simulink model "sschdlexViennaRectifierModel"  (R2026a)
settings: Solver=FixedStepDiscrete  StopTime=0.8  MaxStep=1e-4
PreLoadFcn:
  | % Copyright 2017-2023 The MathWorks, Inc.
  | 
  | %% System Parameters
  | Vs    = 120*sqrt(3); % AC source line-to-line (V, rms)
  | Vpeak = Vs/sqrt(3)*sqrt(2); % AC source line-to-ground (V, peak)
  | R = 0.1;  % Resistance (Ohm)
  | L = 2e-3; % Inductance (H)
  | Vdcnom = 400;  % Nominal output dc voltage (V)
  | Pnom   = 10e3; % Nominal power (W)
  | Imax   = Pnom/(1.5*Vpeak); % Maximum ac current        (A)
  | Inom   = Pnom/Vdcnom;      % Nominal output dc current (A)
  | Iload  = 0.2*Inom;         % Initial load current      (A)
  | 
  | %% Control Parameters
  | fsw = 5e3;        % Switching frequency (Hz)
  | Ts  = 1/(50*fsw); % Fundamental sample time (s)
  | Tsc = 1/(10*fsw); % Control sample time (s)
  | 
  | Kp_vdc = 0.7386; % Proportional gain dc-link voltage controller
  | Ki_vdc = 135.6;  % Integral gain dc-link voltage controller
  | Kp_id  = 8.407;  % Proportional gain d-axis current controller
  | Ki_id  = 1127;   % Integral gain d-axis current controller
  | Kp_iq  = 11.91;  % Proportional gain q-axis current controller
  | Ki_iq  = 3706;   % Integral gain q-axis current controller
  | Kp_vn  = 0.4912; % Proportional gain neutral voltage controller
libraries: ee_lib x27, nesl_utility x13, fl_lib x10, eeTransforms x4, slpidlib x4, eeGeneralControl x4, eePwmGeneratorViennaRectifier x1, eeSinusoidalMeasurement x1, eePowerMeasurement x1
(part 1 of 2)
CloseFcn:
  | try,close(h1_ee_vienna_rectifier),end
  | clear h1_ee_vienna_rectifier
  | 
  | clear simlog_ee_vienna_rectifier
  | clear logsout_ee_vienna_rectifier
  | 
  | clear Vs Vpeak R L Vdcnom Pnom Imax Inom Iload
  | clear fsw Ts Tsc Kp_vdc Ki_vdc Kp_id Ki_id Kp_iq Ki_iq Kp_vn
Description:
  | Vienna Rectifier Control
settings Model: DataTypeOverride=Off  Creator=The MathWorks, Inc.  LastModifiedBy=The MathWorks, Inc.
settings DataIOCC: SignalLoggingName=logsout_ee_vienna_rectifier
settings OptimizationCC: ConditionallyExecuteInputs=off
settings DebuggingCC: AlgebraicLoopMsg=error  UnderspecifiedInitializationDetection=Classic  SingleTaskRateTransMsg=error  PregeneratedLibrarySubsystemCodeDiagnostic=none
settings HardwareCC: ProdHWDeviceType=ASIC/FPGA->ASIC/FPGA  TargetBitPerLong=64.0  TargetBitPerPointer=64.0  TargetBitPerSizeT=64.0  TargetBitPerPtrDiffT=64.0  TargetLongLongMode=on  TargetIntDivRoundTo=Zero  TargetEndianess=LittleEndian  TargetWordSize=64.0  TargetHWDeviceType=Custom Processor->MATLAB Host Computer  ProdEqTarget=off
settings SimscapeCC: SimscapeNormalizeSystem=off  SimscapeNominalValues="[{\"value\":\"1\",\"unit\":\"A\"},{\"value\":\"1\",\"unit\":\"bar\"},{\"value\":\"1\",\"unit\":\"cm^2\"},{\"value\":\"1\",\"unit\":\"cm^3/s\"},{\"value\":\"1\",\"unit\":\"kJ/kg\"},{\"value\":\"1\",\"unit\":\"kW\"},{\"value\":\"1\",\"unit\":\"l\"},{\"value\":\"1\",\"unit\":\"N\"},{\"value\":\"1\",\"unit\":\"N*m\"},{\"value\":\"1\",\"unit\":\"V\"}]"  SimscapeLogName=simlog_ee_vienna_rectifier  SimscapeLogDataHistory=200000.0

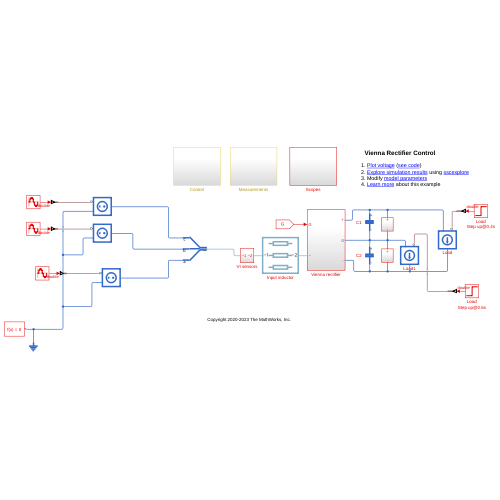
[thumbnail: Simulink's stored preview of the top-level diagram]
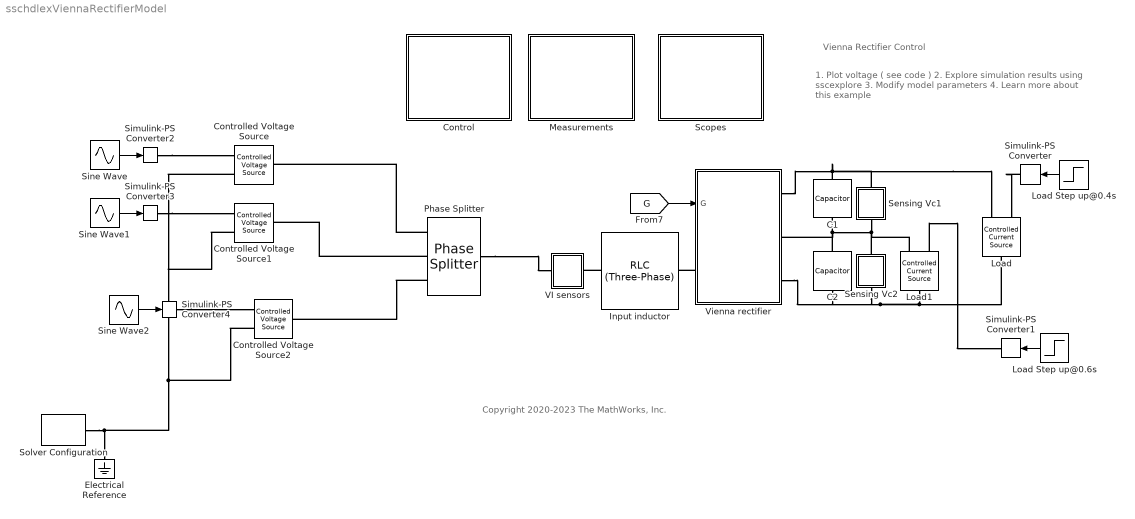
== system sschdlexViennaRectifierModel ==
  note: Copyright 2020-2023 The MathWorks, Inc.
  note: Vienna Rectifier Control
  note: 1. Plot voltage ( see code )
      | 2. Explore simulation results using sscexplore
      | 3. Modify model parameters
      | 4. Learn more about this example
  C1 : fl_lib/Electrical/Electrical Elements/Capacitor  c=2000e-6 F  r=1e-5 Ohm  g=0 1/Ohm  i_specify=off  i_priority=None  i=0 A  i_nominal_specify=off  i_nominal_value=1  i_nominal_unit=A  v_specify=off  v_priority=None  v=0 V  v_nominal_specify=off  v_nominal_value=1  v_nominal_unit=V  vc_specify=off  vc_priority=High  vc=0 V  vc_nominal_specify=off  vc_nominal_value=1  vc_nominal_unit=V
  C2 : fl_lib/Electrical/Electrical Elements/Capacitor  c=2000e-6 F  r=1e-5 Ohm  g=0 1/Ohm  i_specify=off  i_priority=None  i=0 A  i_nominal_specify=off  i_nominal_value=1  i_nominal_unit=A  v_specify=off  v_priority=None  v=0 V  v_nominal_specify=off  v_nominal_value=1  v_nominal_unit=V  vc_specify=off  vc_priority=High  vc=0 V  vc_nominal_specify=off  vc_nominal_value=1  vc_nominal_unit=V
  Control : Subsystem
  Controlled Voltage Source : fl_lib/Electrical/Electrical Sources/Controlled Voltage Source
  Controlled Voltage Source1 : fl_lib/Electrical/Electrical Sources/Controlled Voltage Source
  Controlled Voltage Source2 : fl_lib/Electrical/Electrical Sources/Controlled Voltage Source
  Electrical Reference : fl_lib/Electrical/Electrical Elements/Electrical Reference
  Input inductor : ee_lib/Passive/RLC Assemblies/RLC (Three-Phase)  port_option=ee.enum.threePhasePort.composite  component_structure=4  R=R Ohm  L=L H  C=1e-6 F  R_parasitic=1e-6 Ohm  G_parasitic=1e-6 1/Ohm  IL_specify=off  IL_priority=High  IL=[ 0 0 0 ] A  IL_nominal_specify=off  IL_nominal_value=1  IL_nominal_unit=A  VC_specify=off  VC_priority=High  VC=[ 0 0 0 ] V  VC_nominal_specify=off  VC_nominal_value=1  VC_nominal_unit=V
  Load : fl_lib/Electrical/Electrical Sources/Controlled Current Source
  Load Step up@0.4s : Step  Time=0.4  InitialValue=Iload  FinalValue=Inom  SampleTime=Ts
  Load Step up@0.6s : Step  Time=0.6  FinalValue=2  SampleTime=Ts
  Load1 : fl_lib/Electrical/Electrical Sources/Controlled Current Source
  Measurements : Subsystem
  Phase Splitter : ee_lib/Connectors & References/Phase Splitter
  Scopes : Subsystem
  Sensing Vc1 : Subsystem
  Sensing Vc2 : Subsystem
  Simulink-PS Converter{,1..4} (5 alike) : nesl_utility/Simulink-PS Converter  PhysicalDomain=network_engine_domain  SubClassName=ps_input  LeftPortType=input  RightPortType=output  PseudoPeriodic=off  Frequencies=[]  NoiseDistribution=none  NoiseParameters=[]  Unit=1  AffineConversion=off  FilteringAndDerivatives=provide  SimscapeFilterOrder=1  InputFilterTimeConstant=0.001  UdotUserProvided=0
  Sine Wave : Sin  Amplitude=Vs/sqrt(2)  Frequency=2*pi*60  Phase=2*pi/3  SampleTime=Ts
  Sine Wave1 : Sin  Amplitude=Vs/sqrt(2)  Frequency=2*pi*60  Phase=4*pi/3  SampleTime=Ts
  Sine Wave2 : Sin  Amplitude=Vs/sqrt(2)  Frequency=2*pi*60  SampleTime=Ts
  Solver Configuration : nesl_utility/Solver Configuration  PhysicalDomain=network_engine_domain  SubClassName=solver  LeftPortType=input  RightPortType=generic  Tones=[]  Harmonics=[]  SimulateNoise=off  Profile=off  UseLocalSampling=off  EnableSwitchedLinearOptims=on  FrequencyDomain=off  UseCCode=off  RelTol=0.001  AbsTol=1e-06  MinStep=1e-09  ToWorkspace=off  RevertToSquareIcSolve=off  NumHomotopyIterations=100  PhasorMode=off  PhasorModeNumHarmonics=1  ConsistencySolver=NEWTON_FTOL  CanonicalOrdering=UNORDERED  OptimizeIntermediates=UNOPTIMIZED  IndexReductionMethod=DerivativeReplacement  DoDC=off  ResidualTolerance=1e-09  ConsistencyTolSource=GLOBAL  ConsistencyAbsTol=0.001  ConsistencyRelTol=0.001  ConsistencyTolFactor=0.001  UseLocalSolver=on  LocalSolverChoice=NE_BACKWARD_EULER_ADVANCER  ResolveIndetEquations=on  FunctionEvalNumThread=1  LocalSolverSampleTime=Ts  DoFixedCost=off  MaxNonlinIter=4  MaxModeIter=2  ComputeImpulses=off  ImpulseIterations=2  LinearAlgebra=auto  LinearAlgebraNumThread=0  EquationFormulation=NE_TIME_EF  DelaysMemoryBudget=1024  AutomaticFiltering=on  FilteringTimeConstant=0.001  PartitionStorageMethod=AS_NEEDED  PartitionMemoryBudget=1024  PartitionMethod=FAST  MultibodyUseLocalSolver=off  MultibodyLocalSolverChoice=ODE1  MultibodyLocalSolverSampleTime=0.001
  VI sensors : Subsystem
  Vienna rectifier : Subsystem
  wires:
  Load Step up@0.4s/1 -> Simulink-PS Converter/1
  [G] -> Vienna rectifier/1(G)
  Load Step up@0.6s/1 -> Simulink-PS Converter1/1
  Sine Wave/1 -> Simulink-PS Converter2/1
  Sine Wave1/1 -> Simulink-PS Converter3/1
  Sine Wave2/1 -> Simulink-PS Converter4/1
  connections:
  C1/RConn1 -- C2/LConn1 -- Vienna rectifier/RConn2 -- Load1/RConn2 -- Sensing Vc2/LConn1 -- Sensing Vc1/RConn1
  Vienna rectifier/RConn1 -- C1/LConn1 -- Sensing Vc1/LConn1 -- Load/RConn2
  Solver Configuration/RConn1 -- Controlled Voltage Source2/RConn2 -- Controlled Voltage Source1/RConn2 -- Controlled Voltage Source/RConn2 -- Electrical Reference/LConn1
  Sensing Vc2/RConn1 -- C2/RConn1 -- Vienna rectifier/RConn3 -- Load1/LConn1 -- Load/LConn1
  Phase Splitter/LConn1 -- VI sensors/LConn1
  Simulink-PS Converter/RConn1 -- Load/RConn1
  Input inductor/LConn1 -- VI sensors/RConn1
  Vienna rectifier/LConn1 -- Input inductor/RConn1
  Load1/RConn1 -- Simulink-PS Converter1/RConn1
  Simulink-PS Converter2/RConn1 -- Controlled Voltage Source/RConn1
  Simulink-PS Converter3/RConn1 -- Controlled Voltage Source1/RConn1
  Simulink-PS Converter4/RConn1 -- Controlled Voltage Source2/RConn1
  Phase Splitter/RConn3 -- Controlled Voltage Source/LConn1
  Phase Splitter/RConn2 -- Controlled Voltage Source1/LConn1
  Phase Splitter/RConn1 -- Controlled Voltage Source2/LConn1

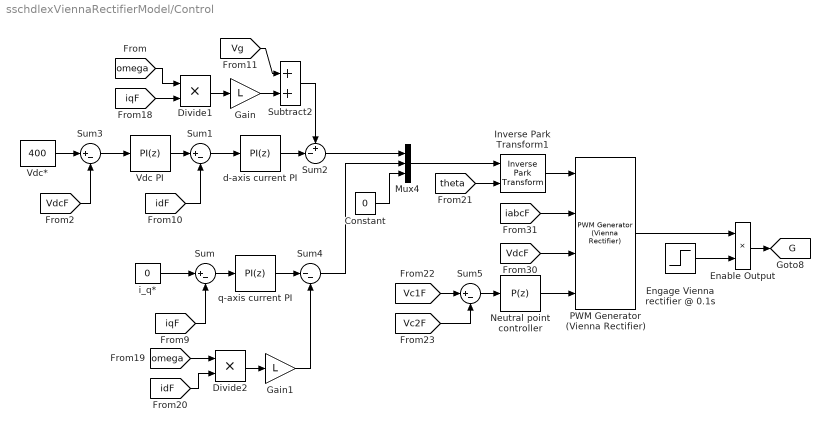
== system sschdlexViennaRectifierModel/Control ==
  Constant : Constant  Value=0  SampleTime=Tsc
  Divide1 : Product  Inputs=**
  Divide2 : Product  Inputs=**
  Enable Output : Product
  Engage Vienna rectifier @ 0.1s : Step  Time=0.1  SampleTime=Ts
  Gain : Gain  Gain=L
  Gain1 : Gain  Gain=L
  Inverse Park Transform1 : eeTransforms/Inverse Park Transform  AxisAlignment=Q-axis  PowerInvariant=off
  Mux4 : Mux  Inputs=3
  Neutral point controller : slpidlib/PID Controller  Controller=P  Form=Parallel  TimeDomain=Discrete-time  UseExternalTs=off  SampleTime=-1  IntegratorMethod=Forward Euler  FilterMethod=Forward Euler  ControllerParametersSource=internal  P=Kp_vn  I=80/2  UseKiTs=off  D=0  UseExternalDerivativeSource=off  N=100  UseFilter=on  TunerSelectOption=Transfer Function Based (PID Tuner App)  InitialConditionSource=internal  InitialConditionForIntegrator=0  InitialConditionForFilter=0  DifferentiatorICPrevScaledInput=0  ExternalReset=none  TrackingMode=off  Kt=1  LimitOutput=on  SatLimitsSource=internal  UpperSaturationLimit=1  LowerSaturationLimit=-1  LinearizeAsGain=on  AntiWindupMode=back-calculation  Kb=1000  LimitIntegrator=off  UpperIntegratorSaturationLimit=inf  LowerIntegratorSaturationLimit=-inf  POutMin=[]  POutMax=[]  IOutMin=[]  IOutMax=[]  DOutMin=[]  DOutMax=[]  NOutMin=[]  NOutMax=[]  SumOutMin=[]  SumOutMax=[]  SaturationOutMin=[]  SaturationOutMax=[]  PParamMin=[]  PParamMax=[]  IParamMin=[]  IParamMax=[]  DParamMin=[]  DParamMax=[]  NParamMin=[]  NParamMax=[]  KbParamMin=[]  KbParamMax=[]  KtParamMin=[]  KtParamMax=[]  KbOutMin=[]  KbOutMax=[]  KtOutMin=[]  KtOutMax=[]  IntegratorOutMin=[]  IntegratorOutMax=[]  FilterOutMin=[]  FilterOutMax=[]  SumI1OutMin=[]  SumI1OutMax=[]  SumI2OutMin=[]  SumI2OutMax=[]  SumI3OutMin=[]  SumI3OutMax=[]  SumI4OutMin=[]  SumI4OutMax=[]  SumDOutMin=[]  SumDOutMax=[]  DifferentiatorOutMin=[]  DifferentiatorOutMax=[]  FilterDiffOutCoefMin=[]  FilterDiffOutCoefMax=[]  ReciprocalOutMin=[]  ReciprocalOutMax=[]  SumDenOutMin=[]  SumDenOutMax=[]  SumNumOutMin=[]  SumNumOutMax=[]  DivideOutMin=[]  DivideOutMax=[]  UdiffTsProdOutMin=[]  UdiffTsProdOutMax=[]  NTsProdOutMin=[]  NTsProdOutMax=[]  UintegralTsProdOutMin=[]  UintegralTsProdOutMax=[]  UngainTsProdOutMin=[]  UngainTsProdOutMax=[]  ClampingZeroOutDataTypeStr=Inherit: Inherit via back propagation  ClampingZeroOutMin=[]  ClampingZeroOutMax=[]  FilterDenConstantOutDataTypeStr=Inherit: Inherit via back propagation  FilterDenConstantOutMin=[]  FilterDenConstantOutMax=[]  PCopyOutDataTypeStr=Inherit: Inherit via back propagation  PCopyOutMin=[]  PCopyOutMax=[]  NCopyOutDataTypeStr=Inherit: Inherit via back propagation  NCopyOutMin=[]  NCopyOutMax=[]  IntegratorContinuousStateAttributes=''  IntegratorStateMustResolveToSignalObject=off  IntegratorRTWStateStorageClass=Auto  FilterContinuousStateAttributes=''  FilterStateMustResolveToSignalObject=off  FilterRTWStateStorageClass=Auto  ParallelPVariant=InternalParameters  IdealPVariant=Disabled  IVariant=Disabled  DVariant=Disabled  IntegratorVariant=Disabled  SatVariant=Enabled  AWVariant=Disabled  PCopyVariant=Disabled  TRVariant=Disabled  FdbkBlocksVariant=Forward  IdealPFdbkVariant=Disabled  SatFdbkVariant=Disabled  DerivativeFilterVariant=Disabled  NVariant=Disabled  NCopyVariant=Disabled_SignalSpec  FilterICVariant=Disabled  IntegratorICVariant=Disabled  ExternalResetVariant=Disabled  TRSumVariant=Passthrough  SumFdbkVariant=Disabled  SumVariant=Passthrough_P  TsampFilterVariant=InternalTs  TsampNgainVariant=Passthrough  TsampIntegralVariant=Disabled_SignalSpec  ExternalSaturationOutDataTypeStr=Inherit: Same as second input  DerivativeSourceVariant=Disabled  PreIntVariant=InternalPreInt
  PWM Generator (Vienna Rectifier) : eePwmGeneratorViennaRectifier/PWM Generator (Vienna Rectifier)  fsw=fsw  Ts=Ts
      settings: SamplingMode=Asymmetric
  Subtract2 : Sum
  Sum{,1,3,5} (4 alike) : Sum  Inputs=|+-
  Sum2 : Sum  Inputs=+-|
  Sum4 : Sum  Inputs=|--
  Vdc PI : slpidlib/PID Controller  Controller=PI  Form=Parallel  TimeDomain=Discrete-time  UseExternalTs=off  SampleTime=Tsc  IntegratorMethod=Forward Euler  FilterMethod=Forward Euler  ControllerParametersSource=internal  P=Kp_vdc  I=Ki_vdc  UseKiTs=off  D=0  UseExternalDerivativeSource=off  N=100  UseFilter=on  TunerSelectOption=Transfer Function Based (PID Tuner App)  InitialConditionSource=internal  InitialConditionForIntegrator=0  InitialConditionForFilter=0  DifferentiatorICPrevScaledInput=0  ExternalReset=none  TrackingMode=off  Kt=1  LimitOutput=on  SatLimitsSource=internal  UpperSaturationLimit=1.5*Imax  LowerSaturationLimit=-1.5*Imax  LinearizeAsGain=on  AntiWindupMode=back-calculation  Kb=1000  LimitIntegrator=off  UpperIntegratorSaturationLimit=inf  LowerIntegratorSaturationLimit=-inf  POutMin=[]  POutMax=[]  IOutMin=[]  IOutMax=[]  DOutMin=[]  DOutMax=[]  NOutMin=[]  NOutMax=[]  SumOutMin=[]  SumOutMax=[]  SaturationOutMin=[]  SaturationOutMax=[]  PParamMin=[]  PParamMax=[]  IParamMin=[]  IParamMax=[]  DParamMin=[]  DParamMax=[]  NParamMin=[]  NParamMax=[]  KbParamMin=[]  KbParamMax=[]  KtParamMin=[]  KtParamMax=[]  KbOutMin=[]  KbOutMax=[]  KtOutMin=[]  KtOutMax=[]  IntegratorOutMin=[]  IntegratorOutMax=[]  FilterOutMin=[]  FilterOutMax=[]  SumI1OutMin=[]  SumI1OutMax=[]  SumI2OutMin=[]  SumI2OutMax=[]  SumI3OutMin=[]  SumI3OutMax=[]  SumI4OutMin=[]  SumI4OutMax=[]  SumDOutMin=[]  SumDOutMax=[]  DifferentiatorOutMin=[]  DifferentiatorOutMax=[]  FilterDiffOutCoefMin=[]  FilterDiffOutCoefMax=[]  ReciprocalOutMin=[]  ReciprocalOutMax=[]  SumDenOutMin=[]  SumDenOutMax=[]  SumNumOutMin=[]  SumNumOutMax=[]  DivideOutMin=[]  DivideOutMax=[]  UdiffTsProdOutMin=[]  UdiffTsProdOutMax=[]  NTsProdOutMin=[]  NTsProdOutMax=[]  UintegralTsProdOutMin=[]  UintegralTsProdOutMax=[]  UngainTsProdOutMin=[]  UngainTsProdOutMax=[]  ClampingZeroOutDataTypeStr=Inherit: Inherit via back propagation  ClampingZeroOutMin=[]  ClampingZeroOutMax=[]  FilterDenConstantOutDataTypeStr=Inherit: Inherit via back propagation  FilterDenConstantOutMin=[]  FilterDenConstantOutMax=[]  PCopyOutDataTypeStr=Inherit: Inherit via back propagation  PCopyOutMin=[]  PCopyOutMax=[]  NCopyOutDataTypeStr=Inherit: Inherit via back propagation  NCopyOutMin=[]  NCopyOutMax=[]  IntegratorContinuousStateAttributes=''  IntegratorStateMustResolveToSignalObject=off  IntegratorRTWStateStorageClass=Auto  FilterContinuousStateAttributes=''  FilterStateMustResolveToSignalObject=off  FilterRTWStateStorageClass=Auto  ParallelPVariant=InternalParameters  IdealPVariant=Disabled  IVariant=InternalParameters  DVariant=Disabled  IntegratorVariant=Discrete  SatVariant=Enabled  AWVariant=BackCalculation  PCopyVariant=Disabled  TRVariant=Disabled  FdbkBlocksVariant=Forward  IdealPFdbkVariant=Disabled  SatFdbkVariant=Disabled  DerivativeFilterVariant=Disabled  NVariant=Disabled  NCopyVariant=Disabled_SignalSpec  FilterICVariant=Disabled  IntegratorICVariant=InternalICs  ExternalResetVariant=Disabled  TRSumVariant=Passthrough  SumFdbkVariant=Disabled  SumVariant=Sum_PI  TsampFilterVariant=InternalTs  TsampNgainVariant=Passthrough  TsampIntegralVariant=Disabled_SignalSpec  ExternalSaturationOutDataTypeStr=Inherit: Same as second input  DerivativeSourceVariant=Disabled  PreIntVariant=InternalPreInt
  Vdc* : Constant  Value=400  SampleTime=Tsc
  d-axis current PI : slpidlib/PID Controller  Controller=PI  Form=Parallel  TimeDomain=Discrete-time  UseExternalTs=off  SampleTime=Tsc  IntegratorMethod=Forward Euler  FilterMethod=Forward Euler  ControllerParametersSource=internal  P=Kp_id  I=Ki_id  UseKiTs=off  D=0  UseExternalDerivativeSource=off  N=100  UseFilter=on  TunerSelectOption=Transfer Function Based (PID Tuner App)  InitialConditionSource=internal  InitialConditionForIntegrator=0  InitialConditionForFilter=0  DifferentiatorICPrevScaledInput=0  ExternalReset=none  TrackingMode=off  Kt=1  LimitOutput=on  SatLimitsSource=internal  UpperSaturationLimit=R*Imax*2  LowerSaturationLimit=-R*Imax*2  LinearizeAsGain=on  AntiWindupMode=back-calculation  Kb=1000  LimitIntegrator=off  UpperIntegratorSaturationLimit=inf  LowerIntegratorSaturationLimit=-inf  POutMin=[]  POutMax=[]  IOutMin=[]  IOutMax=[]  DOutMin=[]  DOutMax=[]  NOutMin=[]  NOutMax=[]  SumOutMin=[]  SumOutMax=[]  SaturationOutMin=[]  SaturationOutMax=[]  PParamMin=[]  PParamMax=[]  IParamMin=[]  IParamMax=[]  DParamMin=[]  DParamMax=[]  NParamMin=[]  NParamMax=[]  KbParamMin=[]  KbParamMax=[]  KtParamMin=[]  KtParamMax=[]  KbOutMin=[]  KbOutMax=[]  KtOutMin=[]  KtOutMax=[]  IntegratorOutMin=[]  IntegratorOutMax=[]  FilterOutMin=[]  FilterOutMax=[]  SumI1OutMin=[]  SumI1OutMax=[]  SumI2OutMin=[]  SumI2OutMax=[]  SumI3OutMin=[]  SumI3OutMax=[]  SumI4OutMin=[]  SumI4OutMax=[]  SumDOutMin=[]  SumDOutMax=[]  DifferentiatorOutMin=[]  DifferentiatorOutMax=[]  FilterDiffOutCoefMin=[]  FilterDiffOutCoefMax=[]  ReciprocalOutMin=[]  ReciprocalOutMax=[]  SumDenOutMin=[]  SumDenOutMax=[]  SumNumOutMin=[]  SumNumOutMax=[]  DivideOutMin=[]  DivideOutMax=[]  UdiffTsProdOutMin=[]  UdiffTsProdOutMax=[]  NTsProdOutMin=[]  NTsProdOutMax=[]  UintegralTsProdOutMin=[]  UintegralTsProdOutMax=[]  UngainTsProdOutMin=[]  UngainTsProdOutMax=[]  ClampingZeroOutDataTypeStr=Inherit: Inherit via back propagation  ClampingZeroOutMin=[]  ClampingZeroOutMax=[]  FilterDenConstantOutDataTypeStr=Inherit: Inherit via back propagation  FilterDenConstantOutMin=[]  FilterDenConstantOutMax=[]  PCopyOutDataTypeStr=Inherit: Inherit via back propagation  PCopyOutMin=[]  PCopyOutMax=[]  NCopyOutDataTypeStr=Inherit: Inherit via back propagation  NCopyOutMin=[]  NCopyOutMax=[]  IntegratorContinuousStateAttributes=''  IntegratorStateMustResolveToSignalObject=off  IntegratorRTWStateStorageClass=Auto  FilterContinuousStateAttributes=''  FilterStateMustResolveToSignalObject=off  FilterRTWStateStorageClass=Auto  ParallelPVariant=InternalParameters  IdealPVariant=Disabled  IVariant=InternalParameters  DVariant=Disabled  IntegratorVariant=Discrete  SatVariant=Enabled  AWVariant=BackCalculation  PCopyVariant=Disabled  TRVariant=Disabled  FdbkBlocksVariant=Forward  IdealPFdbkVariant=Disabled  SatFdbkVariant=Disabled  DerivativeFilterVariant=Disabled  NVariant=Disabled  NCopyVariant=Disabled_SignalSpec  FilterICVariant=Disabled  IntegratorICVariant=InternalICs  ExternalResetVariant=Disabled  TRSumVariant=Passthrough  SumFdbkVariant=Disabled  SumVariant=Sum_PI  TsampFilterVariant=InternalTs  TsampNgainVariant=Passthrough  TsampIntegralVariant=Disabled_SignalSpec  ExternalSaturationOutDataTypeStr=Inherit: Same as second input  DerivativeSourceVariant=Disabled  PreIntVariant=InternalPreInt
  i_q* : Constant  Value=0  SampleTime=Tsc
  q-axis current PI : slpidlib/PID Controller  Controller=PI  Form=Parallel  TimeDomain=Discrete-time  UseExternalTs=off  SampleTime=Tsc  IntegratorMethod=Forward Euler  FilterMethod=Forward Euler  ControllerParametersSource=internal  P=Kp_iq  I=Ki_iq  UseKiTs=off  D=0  UseExternalDerivativeSource=off  N=100  UseFilter=on  TunerSelectOption=Transfer Function Based (PID Tuner App)  InitialConditionSource=internal  InitialConditionForIntegrator=0  InitialConditionForFilter=0  DifferentiatorICPrevScaledInput=0  ExternalReset=none  TrackingMode=off  Kt=1  LimitOutput=on  SatLimitsSource=internal  UpperSaturationLimit=R*Imax*2  LowerSaturationLimit=-R*Imax*2  LinearizeAsGain=on  AntiWindupMode=back-calculation  Kb=1000  LimitIntegrator=off  UpperIntegratorSaturationLimit=inf  LowerIntegratorSaturationLimit=-inf  POutMin=[]  POutMax=[]  IOutMin=[]  IOutMax=[]  DOutMin=[]  DOutMax=[]  NOutMin=[]  NOutMax=[]  SumOutMin=[]  SumOutMax=[]  SaturationOutMin=[]  SaturationOutMax=[]  PParamMin=[]  PParamMax=[]  IParamMin=[]  IParamMax=[]  DParamMin=[]  DParamMax=[]  NParamMin=[]  NParamMax=[]  KbParamMin=[]  KbParamMax=[]  KtParamMin=[]  KtParamMax=[]  KbOutMin=[]  KbOutMax=[]  KtOutMin=[]  KtOutMax=[]  IntegratorOutMin=[]  IntegratorOutMax=[]  FilterOutMin=[]  FilterOutMax=[]  SumI1OutMin=[]  SumI1OutMax=[]  SumI2OutMin=[]  SumI2OutMax=[]  SumI3OutMin=[]  SumI3OutMax=[]  SumI4OutMin=[]  SumI4OutMax=[]  SumDOutMin=[]  SumDOutMax=[]  DifferentiatorOutMin=[]  DifferentiatorOutMax=[]  FilterDiffOutCoefMin=[]  FilterDiffOutCoefMax=[]  ReciprocalOutMin=[]  ReciprocalOutMax=[]  SumDenOutMin=[]  SumDenOutMax=[]  SumNumOutMin=[]  SumNumOutMax=[]  DivideOutMin=[]  DivideOutMax=[]  UdiffTsProdOutMin=[]  UdiffTsProdOutMax=[]  NTsProdOutMin=[]  NTsProdOutMax=[]  UintegralTsProdOutMin=[]  UintegralTsProdOutMax=[]  UngainTsProdOutMin=[]  UngainTsProdOutMax=[]  ClampingZeroOutDataTypeStr=Inherit: Inherit via back propagation  ClampingZeroOutMin=[]  ClampingZeroOutMax=[]  FilterDenConstantOutDataTypeStr=Inherit: Inherit via back propagation  FilterDenConstantOutMin=[]  FilterDenConstantOutMax=[]  PCopyOutDataTypeStr=Inherit: Inherit via back propagation  PCopyOutMin=[]  PCopyOutMax=[]  NCopyOutDataTypeStr=Inherit: Inherit via back propagation  NCopyOutMin=[]  NCopyOutMax=[]  IntegratorContinuousStateAttributes=''  IntegratorStateMustResolveToSignalObject=off  IntegratorRTWStateStorageClass=Auto  FilterContinuousStateAttributes=''  FilterStateMustResolveToSignalObject=off  FilterRTWStateStorageClass=Auto  ParallelPVariant=InternalParameters  IdealPVariant=Disabled  IVariant=InternalParameters  DVariant=Disabled  IntegratorVariant=Discrete  SatVariant=Enabled  AWVariant=BackCalculation  PCopyVariant=Disabled  TRVariant=Disabled  FdbkBlocksVariant=Forward  IdealPFdbkVariant=Disabled  SatFdbkVariant=Disabled  DerivativeFilterVariant=Disabled  NVariant=Disabled  NCopyVariant=Disabled_SignalSpec  FilterICVariant=Disabled  IntegratorICVariant=InternalICs  ExternalResetVariant=Disabled  TRSumVariant=Passthrough  SumFdbkVariant=Disabled  SumVariant=Sum_PI  TsampFilterVariant=InternalTs  TsampNgainVariant=Passthrough  TsampIntegralVariant=Disabled_SignalSpec  ExternalSaturationOutDataTypeStr=Inherit: Same as second input  DerivativeSourceVariant=Disabled  PreIntVariant=InternalPreInt
  tag scope: G=global
  wires:
  Gain1/1 -> Sum4/2
  Divide2/1 -> Gain1/1
  PWM Generator (Vienna Rectifier)/1 -> Enable Output/1
  [iqF] -> Sum/2
  [Vc1F] -> Sum5/1
  Sum3/1 -> Vdc PI/1
  d-axis current PI/1 -> Sum2/2
  Sum5/1 -> Neutral point controller/1
  Vdc*/1 -> Sum3/1
  Subtract2/1 -> Sum2/1
  [VdcF] -> Sum3/2
  Sum1/1 -> d-axis current PI/1
  Constant/1 -> Mux4/3
  [Vg] -> Subtract2/1
  [idF] -> Divide2/2
  Sum4/1 -> Mux4/2
  i_q*/1 -> Sum/1
  Sum2/1 -> Mux4/1
  [iabcF] -> PWM Generator (Vienna Rectifier)/2
  [VdcF] -> PWM Generator (Vienna Rectifier)/3
  Gain/1 -> Subtract2/2
  Vdc PI/1 -> Sum1/1
  Sum/1 -> q-axis current PI/1
  [Vc2F] -> Sum5/2
  [theta] -> Inverse Park Transform1/2
  [iqF] -> Divide1/2
  [idF] -> Sum1/2
  q-axis current PI/1 -> Sum4/1
  Inverse Park Transform1/1 -> PWM Generator (Vienna Rectifier)/1
  [omega] -> Divide2/1
  Enable Output/1 -> [G]
  Divide1/1 -> Gain/1
  [omega] -> Divide1/1
  Engage Vienna rectifier @ 0.1s/1 -> Enable Output/2
  Neutral point controller/1 -> PWM Generator (Vienna Rectifier)/4
  Mux4/1 -> Inverse Park Transform1/1

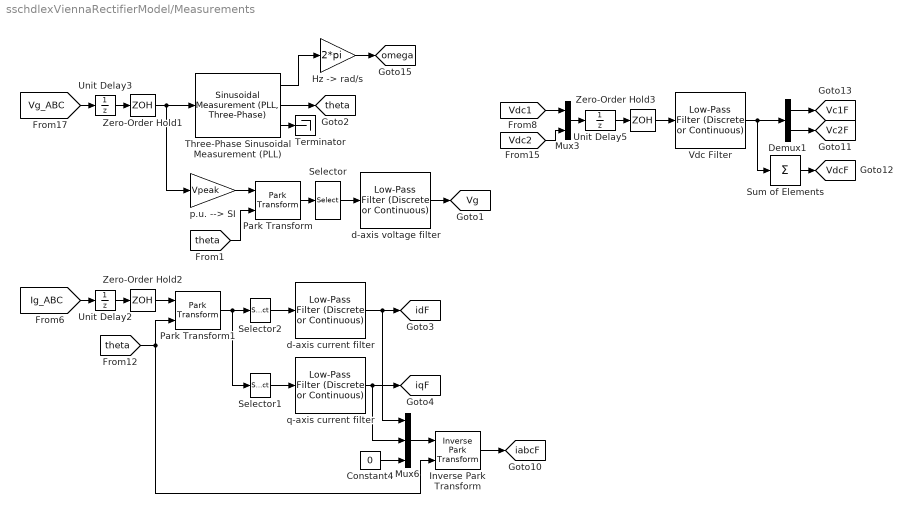
== system sschdlexViennaRectifierModel/Measurements ==
  Constant4 : Constant  Value=0  SampleTime=Tsc
  Demux1 : Demux  Outputs=2
  "Hz -> rad/s" : Gain  Gain=2*pi
  Inverse Park Transform : eeTransforms/Inverse Park Transform  AxisAlignment=Q-axis  PowerInvariant=off
  Mux3 : Mux  Inputs=2
  Mux6 : Mux  Inputs=3
  Park Transform : eeTransforms/Park Transform  AxisAlignment=Q-axis  PowerInvariant=off
  Park Transform1 : eeTransforms/Park Transform  AxisAlignment=Q-axis  PowerInvariant=off
  Selector : Selector  InputPortWidth=3  IndexOptions=Index vector (dialog)  Indices=[1]  OutputSizes=1
  Selector1 : Selector  InputPortWidth=3  IndexOptions=Index vector (dialog)  Indices=[2]  OutputSizes=1
  Selector2 : Selector  InputPortWidth=3  IndexOptions=Index vector (dialog)  Indices=[1]  OutputSizes=1
  Sum of Elements : Sum  Inputs=+
  Terminator : Terminator
  Three-Phase Sinusoidal Measurement (PLL) : eeSinusoidalMeasurement/Sinusoidal Measurement (PLL, Three-Phase)  Kp_LF=200  Ki_LF=2000  F0=60  Theta0=0  Ts=Tsc
  Unit Delay2 : UnitDelay  SampleTime=Ts
  Unit Delay3 : UnitDelay  SampleTime=Ts
  Unit Delay5 : UnitDelay  SampleTime=Ts
  Vdc Filter : eeGeneralControl/Low-Pass Filter (Discrete or Continuous)  K=1  T=5e-4  B=inf  A=-inf  init_option=Inherited from block input  x0=0  Ts=Tsc
  Zero-Order Hold1 : ZeroOrderHold  SampleTime=Tsc
  Zero-Order Hold2 : ZeroOrderHold  SampleTime=Tsc
  Zero-Order Hold3 : ZeroOrderHold  SampleTime=Tsc
  d-axis current filter : eeGeneralControl/Low-Pass Filter (Discrete or Continuous)  K=1  T=5e-4  B=inf  A=-inf  init_option=Inherited from block input  x0=0  Ts=Tsc
  d-axis voltage filter : eeGeneralControl/Low-Pass Filter (Discrete or Continuous)  K=1  T=5e-4  B=inf  A=-inf  init_option=Inherited from block input  x0=0  Ts=Tsc
  "p.u. --> SI " : Gain  Gain=Vpeak
  q-axis current filter : eeGeneralControl/Low-Pass Filter (Discrete or Continuous)  K=1  T=5e-4  B=inf  A=-inf  init_option=Inherited from block input  x0=0  Ts=Tsc
  tag scope: Vc1F=global, Vc2F=global, VdcF=global, Vg=global, iabcF=global, idF=global, iqF=global, omega=global, theta=global
  wires:
  Vdc Filter/1 -> Demux1/1, Sum of Elements/1
  Unit Delay3/1 -> Zero-Order Hold1/1
  Demux1/1 -> [Vc1F]
  Demux1/2 -> [Vc2F]
  Constant4/1 -> Mux6/3
  Unit Delay2/1 -> Zero-Order Hold2/1
  Unit Delay5/1 -> Zero-Order Hold3/1
  Park Transform1/1 -> Selector2/1, Selector1/1
  [Vdc2] -> Mux3/2
  Selector2/1 -> d-axis current filter/1
  Zero-Order Hold1/1 -> Three-Phase Sinusoidal Measurement (PLL)/1, "p.u. --> SI "/1
  "Hz -> rad/s"/1 -> [omega]
  Zero-Order Hold2/1 -> Park Transform1/1
  Sum of Elements/1 -> [VdcF]
  Three-Phase Sinusoidal Measurement (PLL)/1 -> "Hz -> rad/s"/1
  d-axis current filter/1 -> Mux6/1, [idF]
  Mux3/1 -> Unit Delay5/1
  q-axis current filter/1 -> [iqF], Mux6/2
  Mux6/1 -> Inverse Park Transform/1
  Selector1/1 -> q-axis current filter/1
  d-axis voltage filter/1 -> [Vg]
  Zero-Order Hold3/1 -> Vdc Filter/1
  [theta] -> Park Transform1/2, Inverse Park Transform/2
  Inverse Park Transform/1 -> [iabcF]
  Three-Phase Sinusoidal Measurement (PLL)/2 -> [theta]
  [Ig_ABC] -> Unit Delay2/1
  Three-Phase Sinusoidal Measurement (PLL)/3 -> Terminator/1
  Selector/1 -> d-axis voltage filter/1
  [theta] -> Park Transform/2
  [Vg_ABC] -> Unit Delay3/1
  [Vdc1] -> Mux3/1
  "p.u. --> SI "/1 -> Park Transform/1
  Park Transform/1 -> Selector/1

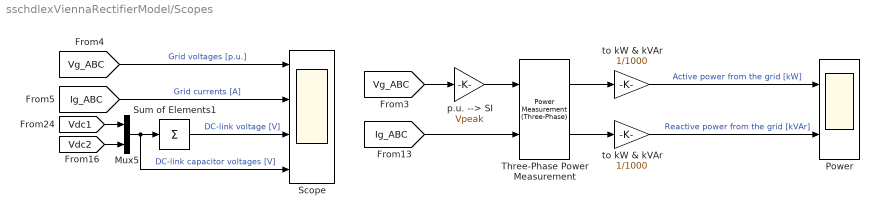
== system sschdlexViennaRectifierModel/Scopes ==
  Mux5 : Mux  Inputs=2
  Power : Scope  NumInputPorts=2
      settings: ActiveDisplayYMinimum=-1.42815  ActiveDisplayYMaximum=12.85331
  Scope : Scope  NumInputPorts=4
      settings: ActiveDisplayYMinimum=-1.53093  ActiveDisplayYMaximum=1.53093
  Sum of Elements1 : Sum  Inputs=+
  Three-Phase Power Measurement : eePowerMeasurement/Power Measurement (Three-Phase)  LabelModeActiveChoice=Discrete  F=60  K=[1]  Seq=Positive  Ts=Ts
  p.u. --> SI : Gain  Gain=Vpeak
  to kW & kVAr : Gain  Gain=1/1000
  "to kW & kVAr " : Gain  Gain=1/1000
  wires:
  [Vdc1] -> Mux5/1
  Three-Phase Power Measurement/1 -> to kW & kVAr/1
  [Vg_ABC] -> Scope/1  "Grid voltages [p.u.]"
  Sum of Elements1/1 -> Scope/3  "DC-link voltage [V]"
  Three-Phase Power Measurement/2 -> "to kW & kVAr "/1
  "to kW & kVAr "/1 -> Power/2  "Reactive power from the grid [kVAr]"
  to kW & kVAr/1 -> Power/1  "Active power from the grid [kW]"
  Mux5/1 -> Scope/4, Sum of Elements1/1  "DC-link capacitor voltages [V]"
  [Vg_ABC] -> p.u. --> SI/1
  [Ig_ABC] -> Three-Phase Power Measurement/2
  [Vdc2] -> Mux5/2
  [Ig_ABC] -> Scope/2  "Grid currents [A]"
  p.u. --> SI/1 -> Three-Phase Power Measurement/1

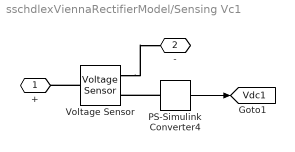
== system sschdlexViennaRectifierModel/Sensing Vc1 ==
  PS-Simulink Converter4 : nesl_utility/PS-Simulink Converter  PhysicalDomain=network_engine_domain  SubClassName=ps_output  LeftPortType=input  RightPortType=output  PseudoPeriodic=off  Frequencies=[]  VectorFormat=1-D array  Unit=V  AffineConversion=off
  Voltage Sensor : fl_lib/Electrical/Electrical Sensors/Voltage Sensor
  + : PMIOPort  Side=Left
  - : PMIOPort  Port=2  Side=Right
  tag scope: Vdc1=global
  wires:
  PS-Simulink Converter4/1 -> [Vdc1]
  connections:
  Voltage Sensor/LConn1 -- +/RConn1
  Voltage Sensor/RConn2 -- -/RConn1
  PS-Simulink Converter4/LConn1 -- Voltage Sensor/RConn1

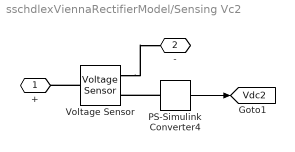
== system sschdlexViennaRectifierModel/Sensing Vc2 ==
  PS-Simulink Converter4 : nesl_utility/PS-Simulink Converter  PhysicalDomain=network_engine_domain  SubClassName=ps_output  LeftPortType=input  RightPortType=output  PseudoPeriodic=off  Frequencies=[]  VectorFormat=1-D array  Unit=V  AffineConversion=off
  Voltage Sensor : fl_lib/Electrical/Electrical Sensors/Voltage Sensor
  + : PMIOPort  Side=Left
  - : PMIOPort  Port=2  Side=Right
  tag scope: Vdc2=global
  wires:
  PS-Simulink Converter4/1 -> [Vdc2]
  connections:
  PS-Simulink Converter4/LConn1 -- Voltage Sensor/RConn1
  Voltage Sensor/RConn2 -- -/RConn1
  Voltage Sensor/LConn1 -- +/RConn1

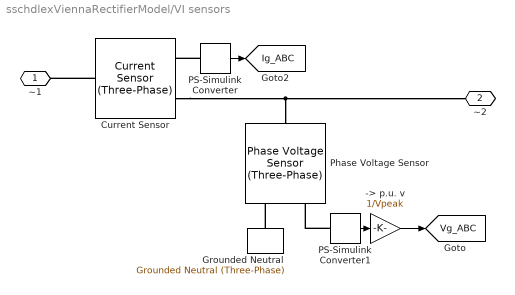
== system sschdlexViennaRectifierModel/VI sensors ==
  -> p.u. v : Gain  Gain=1/Vpeak
  Current Sensor : ee_lib/Sensors & Transducers/Current Sensor (Three-Phase)  port_option=ee.enum.threePhasePort.composite
  Grounded Neutral : ee_lib/Connectors & References/Grounded Neutral (Three-Phase)  port_option=ee.enum.threePhasePort.composite
  PS-Simulink Converter : nesl_utility/PS-Simulink Converter  PhysicalDomain=network_engine_domain  SubClassName=ps_output  LeftPortType=input  RightPortType=output  PseudoPeriodic=off  Frequencies=[]  VectorFormat=1-D array  Unit=1  AffineConversion=off
  PS-Simulink Converter1 : nesl_utility/PS-Simulink Converter  PhysicalDomain=network_engine_domain  SubClassName=ps_output  LeftPortType=input  RightPortType=output  PseudoPeriodic=off  Frequencies=[]  VectorFormat=1-D array  Unit=1  AffineConversion=off
  Phase Voltage Sensor : ee_lib/Sensors & Transducers/Phase Voltage Sensor (Three-Phase)  port_option=ee.enum.threePhasePort.composite
  ~1 : PMIOPort  Side=Left
  ~2 : PMIOPort  Port=2  Side=Right
  tag scope: Ig_ABC=global, Vg_ABC=global
  wires:
  PS-Simulink Converter/1 -> [Ig_ABC]
  PS-Simulink Converter1/1 -> -> p.u. v/1
  -> p.u. v/1 -> [Vg_ABC]
  connections:
  PS-Simulink Converter1/LConn1 -- Phase Voltage Sensor/RConn1
  Current Sensor/RConn2 -- Phase Voltage Sensor/LConn1 -- ~2/RConn1
  PS-Simulink Converter/LConn1 -- Current Sensor/RConn1
  Grounded Neutral/LConn1 -- Phase Voltage Sensor/RConn2
  Current Sensor/LConn1 -- ~1/RConn1
